simulink model "six_lab"  (R2025b)
settings: Solver=VariableStepAuto  StartTime=0.0  StopTime=10.0  RelTol=1e-3
settings Model: Creator=reino  LastModifiedBy=reino

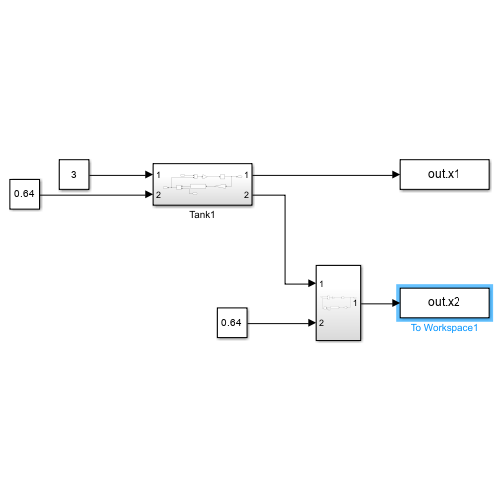
[thumbnail: Simulink's stored preview of the top-level diagram]
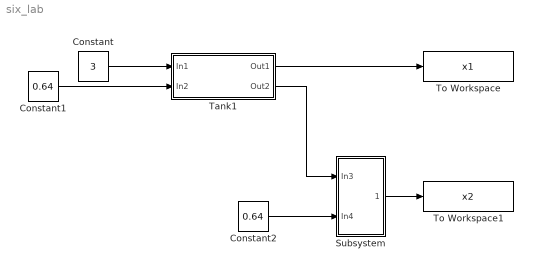
== system six_lab ==
  Constant : Constant  Value=3
  Constant1 : Constant  Value=0.64
  Constant2 : Constant  Value=0.64
  Subsystem : Subsystem
  Tank1 : Subsystem
  To Workspace : ToWorkspace  VariableName=x1  SampleTime=-1
  To Workspace1 : ToWorkspace  VariableName=x2  SampleTime=-1
  wires:
  Tank1/1(Out1) -> To Workspace/1
  Constant1/1 -> Tank1/2(In2)
  Constant/1 -> Tank1/1(In1)
  Subsystem/1(Out1) -> To Workspace1/1
  Constant2/1 -> Subsystem/2(In4)
  Tank1/2(Out2) -> Subsystem/1(In3)

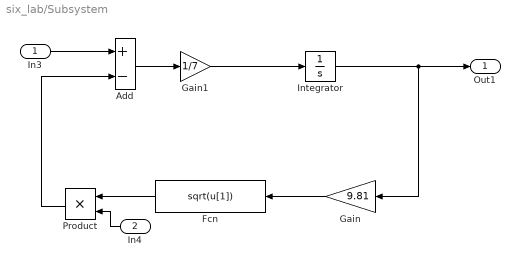
== system six_lab/Subsystem ==
  In3 : Inport
  In4 : Inport  Port=2
  Add : Sum  Inputs=+-
  Fcn : Fcn  Expr=sqrt(u[1])
  Gain : Gain  Gain=9.81
  Gain1 : Gain  Gain=1/7
  Integrator : Integrator  InitialCondition=3
  Product : Product
  Out1 : Outport
  wires:
  In4/1 -> Product/2
  Fcn/1 -> Product/1
  Gain/1 -> Fcn/1
  Gain1/1 -> Integrator/1
  In3/1 -> Add/1
  Add/1 -> Gain1/1
  Product/1 -> Add/2
  Integrator/1 -> Out1/1, Gain/1

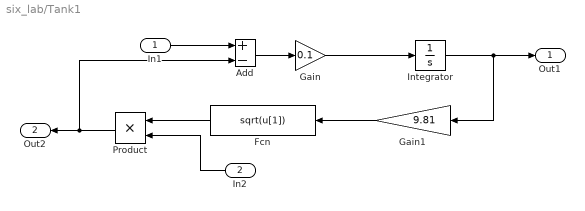
== system six_lab/Tank1 ==
  In1 : Inport
  In2 : Inport  Port=2
  Add : Sum  Inputs=+-
  Fcn : Fcn  Expr=sqrt(u[1])
  Gain : Gain  Gain=0.1
  Gain1 : Gain  Gain=9.81
  Integrator : Integrator  InitialCondition=2
  Product : Product
  Out1 : Outport
  Out2 : Outport  Port=2
  wires:
  Fcn/1 -> Product/1
  Gain1/1 -> Fcn/1
  Integrator/1 -> Out1/1, Gain1/1
  Gain/1 -> Integrator/1
  Add/1 -> Gain/1
  In1/1 -> Add/1
  Product/1 -> Add/2, Out2/1
  In2/1 -> Product/2
